simulink model "modele_freinage_regeneratif_v4"  (R2024a)
settings: Solver=VariableStepAuto  StartTime=0.0  StopTime=40  RelTol=1e-3
libraries: simulink x1
settings Model: Creator=HP  LastModifiedBy=HP

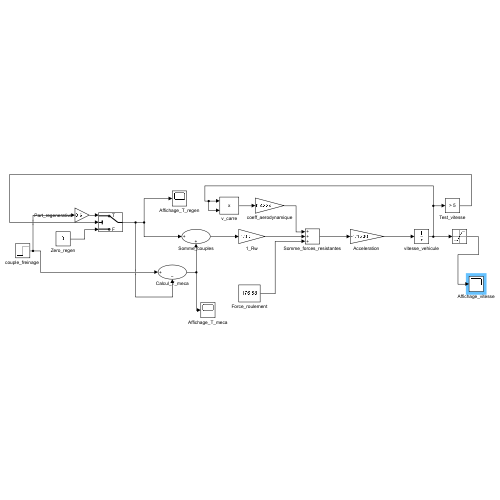
[thumbnail: Simulink's stored preview of the top-level diagram]
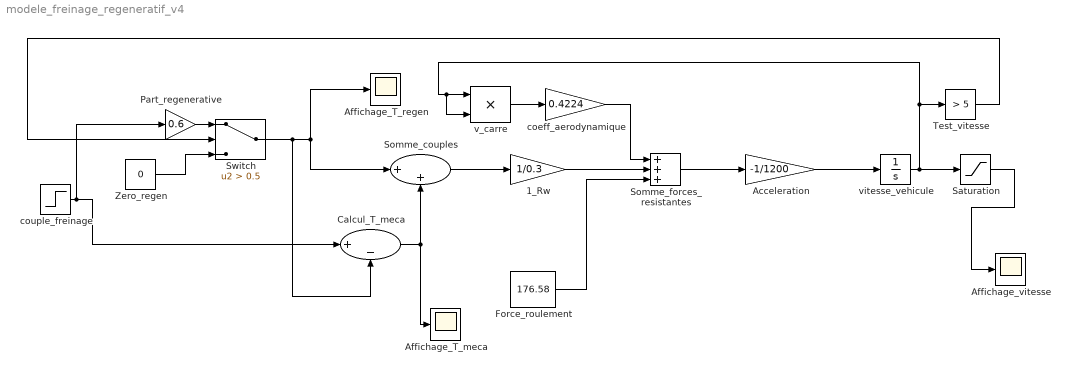
== system modele_freinage_regeneratif_v4 ==
  1_Rw : Gain  Gain=1/0.3
  "Acceleration " : Gain  Gain=-1/1200
  Affichage_T_meca : Scope
  Affichage_T_regen : Scope
  Affichage_vitesse : Scope
  Calcul_T_meca : Sum  Inputs=|+-
  Force_roulement : Constant  Value=176.58
  Part_regenerative : Gain  Gain=0.6
  Saturation : Saturate  UpperLimit=100  LowerLimit=0
  Somme_couples : Sum  Inputs=|++
  Somme_forces_resistantes : Sum  Inputs=+++
  Switch : Switch  Criteria=u2 > Threshold  Threshold=0.5  SaturateOnIntegerOverflow=off  InputSameDT=off
  Test_vitesse : simulink/Logic and Bit Operations/Compare To Constant  relop=>  const=5  OutDataTypeStr=boolean
  Zero_regen : Constant  Value=0
  coeff_aerodynamique : Gain  Gain=0.4224
  "couple_freinage " : Step  After=100  SampleTime=0
  v_carre : Product
  vitesse_vehicule : Integrator  InitialCondition=20
  wires:
  Somme_forces_resistantes/1 -> "Acceleration "/1
  1_Rw/1 -> Somme_forces_resistantes/2
  v_carre/1 -> coeff_aerodynamique/1
  coeff_aerodynamique/1 -> Somme_forces_resistantes/1
  Force_roulement/1 -> Somme_forces_resistantes/3
  vitesse_vehicule/1 -> Saturation/1, Test_vitesse/1, v_carre/2, v_carre/1
  "Acceleration "/1 -> vitesse_vehicule/1
  Saturation/1 -> Affichage_vitesse/1
  "couple_freinage "/1 -> Calcul_T_meca/1, Part_regenerative/1
  Calcul_T_meca/1 -> Somme_couples/2, Affichage_T_meca/1
  Part_regenerative/1 -> Switch/1
  Test_vitesse/1 -> Switch/2
  Zero_regen/1 -> Switch/3
  Switch/1 -> Somme_couples/1, Affichage_T_regen/1, Calcul_T_meca/2
  Somme_couples/1 -> 1_Rw/1
